simulink model "Phugoid"  (R2022a)
settings: Solver=VariableStepAuto  StartTime=0.0  StopTime=0.75  MaxStep=0.01  RelTol=1e-3
undefined symbols (not defined in the file): A, B, C, D, u0
libraries: simulink_extras x1
settings Model: Creator=ks2-parmar  LastModifiedBy=ks2-parmar

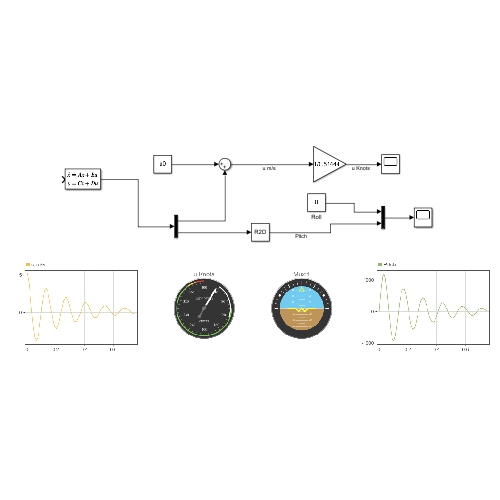
[thumbnail: Simulink's stored preview of the top-level diagram]
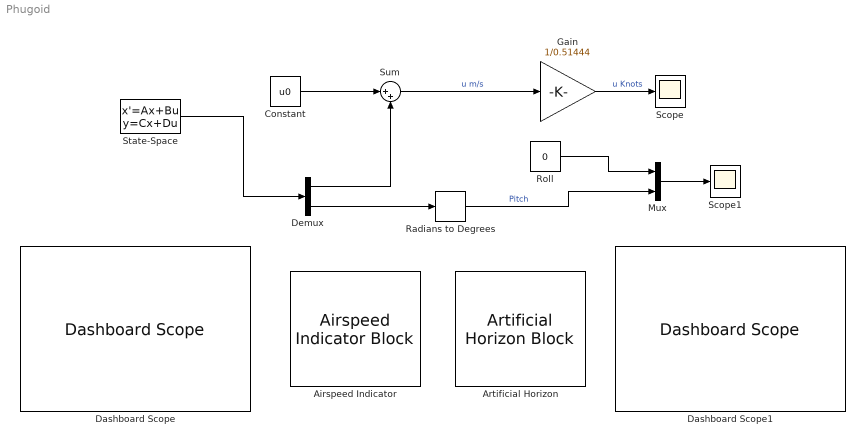
== system Phugoid ==
  Airspeed Indicator : AirspeedIndicatorBlock
  Artificial Horizon : ArtificialHorizonBlock
  Constant : Constant  Value=u0
  Dashboard Scope : DashboardScope
  Dashboard Scope1 : DashboardScope
  Demux : Demux  Outputs=2
  Gain : Gain  Gain=1/0.51444
  Mux : Mux  Inputs=2
  Radians to Degrees : simulink_extras/Transformations/Radians to Degrees
  Roll : Constant  Value=0
  Scope : Scope
  Scope1 : Scope
  State-Space : StateSpace  A=A  B=B  C=C  D=D  InitialCondition=[5;0]
  Sum : Sum  Inputs=|++
  wires:
  State-Space/1 -> Demux/1
  Constant/1 -> Sum/1
  Demux/1 -> Sum/2
  Sum/1 -> Gain/1  "u m/s"
  Gain/1 -> Scope/1  "u Knots"
  Demux/2 -> Radians to Degrees/1
  Radians to Degrees/1 -> Mux/2  "Pitch"
  Roll/1 -> Mux/1
  Mux/1 -> Scope1/1
